simulink model "demoMarinerPathFollowingCourseControl"  (R2024a)
settings: Solver=ode4  StartTime=0.0  StopTime=3000  FixedStep=0.05  RelTol=1e-3  EnableMultiTasking=on
model workspace (MAT data in the model file):
  h_samp = 0.5
libraries: mssSimulink x7, simulink_extras x3
settings Model: Creator=Thor  LastModifiedBy=thor
settings SolverCC: AlgebraicLoopSolver=TrustRegion  AutoInsertRateTranBlk=on
settings DataIOCC: LimitDataPoints=on  SaveFormat=Array  SignalLoggingSaveFormat=ModelDataLogs  ReturnWorkspaceOutputs=off  SignalLoggingName=sigsOut
settings OptimizationCC: BooleanDataType=off  ExpressionDepthLimit=2147483647  InitFltsAndDblsToZero=on  LifeSpan=inf
settings DebuggingCC: SaveWithParameterizedLinksMsg=none  UnderspecifiedInitializationDetection=Classic  MergeDetectMultiDrivingBlocksExec=none  SignalResolutionControl=TryResolveAllWithWarning  MultiTaskDSMMsg=warning  MultiTaskCondExecSysMsg=none  FcnCallInpInsideContextMsg=warning  UnconnectedInputMsg=warning  UnconnectedOutputMsg=warning  UnconnectedLineMsg=warning  StateNameClashWarn=warning  SFUnexpectedBacktrackingDiag=warning  SFNoUnconditionalDefaultTransitionDiag=warning  SFExecutionAtInitializationDiag=none  ArithmeticOperatorsInVariantConditions=warning
settings HardwareCC: ProdBitPerPointer=32  ProdBitPerSizeT=32  ProdBitPerPtrDiffT=32  ProdLargestAtomicFloat=None  ProdIntDivRoundTo=Undefined  ProdEndianess=Unspecified  ProdWordSize=32  ProdHWDeviceType=32-bit Generic  TargetUnknown=on
settings ModelReferenceCC: EnableRefExpFcnMdlSchedulingChecks=on  PropagateSignalLabelsOutOfModel=off
settings SFSimCC: SimUseLocalCustomCode=off  CustomCodeUndefinedFunction=UseInterfaceOnly
settings RTWCC: RTWUseLocalCustomCode=off  GPUComputeCapability=3.5  DLArmComputeVersion=19.05
settings CodeAppCC: StateflowObjectComments=on
settings GRTTargetCC: TargetFcnLib=ansi_tfl_tmw.mat  TargetLangStandard=C89/C90 (ANSI)  ModelReferenceCompliant=off  CombineOutputUpdateFcns=off  MatFileLogging=off  GRTInterface=on
settings ConfigComp: CovMetricSettings=dw  CovSaveCumulativeToWorkspaceVar=on  CovSaveSingleToWorkspaceVar=on  CovExternalEMLEnable=off

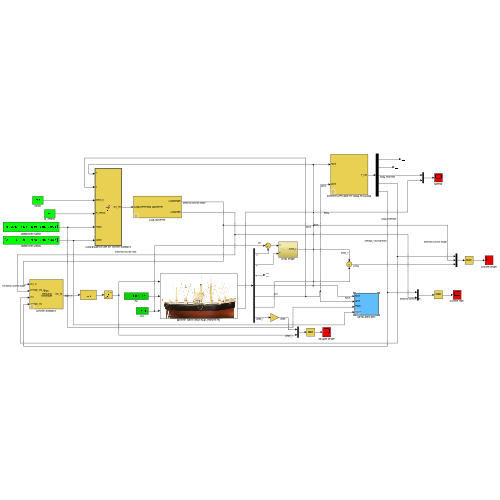
[thumbnail: Simulink's stored preview of the top-level diagram]
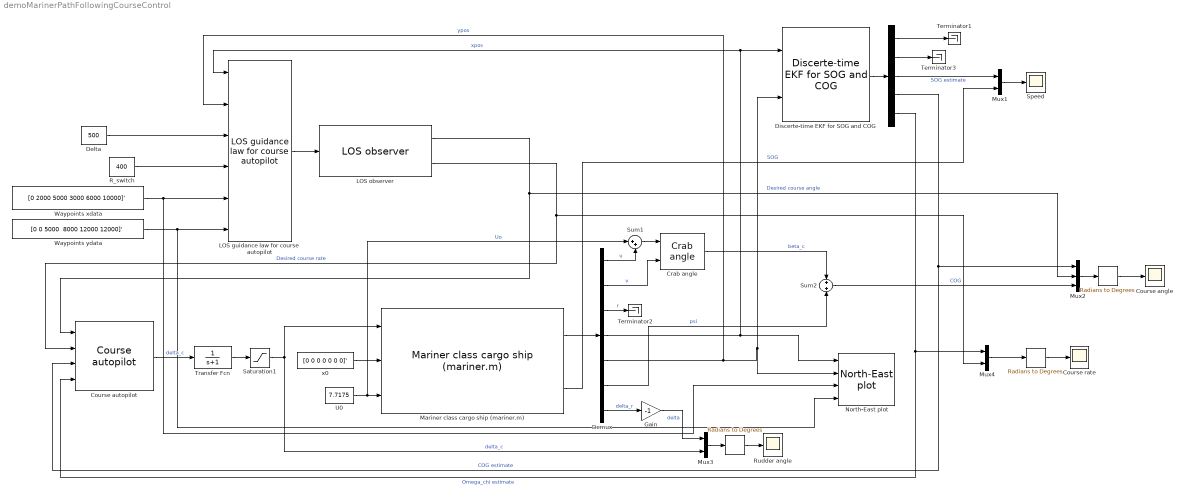
== system demoMarinerPathFollowingCourseControl ==
  "  " : simulink_extras/Transformations/Radians to Degrees
  "      " : simulink_extras/Transformations/Radians to Degrees
  "           " : simulink_extras/Transformations/Radians to Degrees
  "            " : Demux  Outputs=5
  Course angle : Scope
  "Course autopilot " : mssSimulink/Control/Autopilots/Course autopilot   T_nomoto=107.3  K_nomoto=0.185  Kp=1.45  Td=36.27  Ti=200
  "Course rate " : Scope
  Crab angle : mssSimulink/Modelling/Kinematics/Crab angle  SystemSampleTime=-1  VariantActivationTime=update diagram  AllowFlexibleInterface=on  Latency=0  AutoFrameSizeCalculation=off
  Delta : Constant  Value=500
  Demux : Demux  Outputs=7
  Discerte-time EKF for SOG and COG : mssSimulink/Navigation/Estimators/Discerte-time EKF for SOG and COG  alpha_1=0.00001  alpha_2=0.00001  Qd=100*diag([0.1,0.1])  Rd=1000*diag([1 1])  h_samp=0.1
  Gain : Gain  Gain=-1
  LOS guidance law for course autopilot : mssSimulink/Guidance/LOS guidance law for course autopilot  SystemSampleTime=-1  VariantActivationTime=update diagram  AllowFlexibleInterface=on  Latency=0  AutoFrameSizeCalculation=off
  LOS observer : mssSimulink/Guidance/LOS observer  K_f=0.3  alpha=5
  Mariner class cargo ship (mariner.m) : mssSimulink/Marine craft models/Mariner class cargo ship (mariner.m)  SystemSampleTime=-1  VariantActivationTime=update diagram  AllowFlexibleInterface=on  Latency=0  AutoFrameSizeCalculation=off
  Mux1 : Mux  Inputs=2
  Mux2 : Mux  Inputs=3
  Mux3 : Mux  Inputs=2
  Mux4 : Mux  Inputs=2
  North-East plot : mssSimulink/Utilities/Visualization/North-East plot  decimation=10
  R_switch : Constant  Value=400
  Rudder angle : Scope
  Saturation1 : Saturate  UpperLimit=40*pi/180  LowerLimit=-40*pi/180
  Speed : Scope
  Sum1 : Sum  Inputs=|++
  Sum2 : Sum  Inputs=+|+
  Terminator1 : Terminator
  Terminator2 : Terminator
  Terminator3 : Terminator
  Transfer Fcn : TransferFcn  Denominator=[1 1]
  U0 : Constant  Value=7.7175
  Waypoints xdata : Constant  Value=[0 2000 5000 3000 6000 10000]'
  Waypoints ydata : Constant  Value="[0 0 5000  8000 12000 12000]'"
  x0 : Constant  Value=[0 0 0 0 0 0 0]'
  wires:
  "  "/1 -> "Course rate "/1
  "Course autopilot "/1 -> Transfer Fcn/1  "delta_c"
  LOS observer/1 -> "Course autopilot "/1, Mux2/2  "Desired course angle"
  Demux/6 -> Sum2/2  "psi"
  Mariner class cargo ship (mariner.m)/1 -> Demux/1
  U0/1 -> Sum1/1, Mariner class cargo ship (mariner.m)/3  "Uo"
  x0/1 -> Mariner class cargo ship (mariner.m)/2
  Demux/7 -> Gain/1  "delta_r"
  Demux/5 -> LOS guidance law for course autopilot/2, Discerte-time EKF for SOG and COG/2, North-East plot/2  "ypos"
  "           "/1 -> Course angle/1
  "            "/3 -> Mux1/1  "SOG estimate"
  Mux1/1 -> Speed/1
  Mux2/1 -> "           "/1
  Sum2/1 -> Mux2/3  "COG"
  Mux4/1 -> "  "/1
  Mariner class cargo ship (mariner.m)/2 -> Mux1/2  "SOG"
  R_switch/1 -> LOS guidance law for course autopilot/4
  Waypoints ydata/1 -> LOS guidance law for course autopilot/6, North-East plot/4
  Delta/1 -> LOS guidance law for course autopilot/3
  Waypoints xdata/1 -> LOS guidance law for course autopilot/5, North-East plot/3
  "            "/1 -> Terminator1/1
  "            "/2 -> Terminator3/1
  Saturation1/1 -> Mux3/2, Mariner class cargo ship (mariner.m)/1  "delta_c"
  LOS guidance law for course autopilot/1 -> LOS observer/1
  Mux3/1 -> "      "/1
  "            "/5 -> "Course autopilot "/4, Mux4/1  "Omega_chi estimate"
  "            "/4 -> "Course autopilot "/3, Mux2/1  "COG estimate"
  LOS observer/2 -> "Course autopilot "/2, Mux4/2  "Desired course rate"
  Crab angle/1 -> Sum2/1  "beta_c"
  Demux/3 -> Terminator2/1  "r"
  "      "/1 -> Rudder angle/1
  Discerte-time EKF for SOG and COG/1 -> "            "/1
  Demux/4 -> North-East plot/1, Discerte-time EKF for SOG and COG/1, LOS guidance law for course autopilot/1  "xpos"
  Gain/1 -> Mux3/1  "delta"
  Demux/2 -> Crab angle/2  "v"
  Demux/1 -> Sum1/2  "u"
  Sum1/1 -> Crab angle/1
  Transfer Fcn/1 -> Saturation1/1
